simulink model "gm_HFMA_4B_1_5_9_13"  (R2026b)
settings: Solver=FixedStepDiscrete  StopTime=stopTime  FixedStep=1.953125e-06
PreLoadFcn:
  | load('a_luts.mat')
undefined symbols (not defined in the file or in its folder): Ts
libraries: simulink x202, simulink_need_slupdate x99, hdlsllib x91
(part 18 of 20)

== system gm_HFMA_4B_1_5_9_13/Subsystem/HFMA1/crp_temp_shared6/Serializer_Subnetwork1 ==
  in0 : Inport  OutDataTypeStr=fixdt(1,18,0,'DataTypeOverride', 'Off')  PortDimensions=[16]  SampleTime=1.953125e-06
  in1 : Inport  Port=2  OutDataTypeStr=fixdt(0,4,0,'DataTypeOverride', 'Off')  PortDimensions=1  SampleTime=1.953125e-06
  ratechange_splitcomp : Demux  Outputs=16
  splitcomp_multiport : MultiPortSwitch  DataPortOrder=Zero-based contiguous  Inputs=16  DiagnosticForDefault=None  zeroidx=on  OutDataTypeStr=fixdt(1, 18, 0)  SampleTime=1.953125e-06  SaturateOnIntegerOverflow=off  InputSameDT=off
  out0 : Outport  OutDataTypeStr=fixdt(1,18,0,'DataTypeOverride', 'Off')  PortDimensions=1  SampleTime=1.953125e-06
  wires:
  in0/1 -> ratechange_splitcomp/1
  in1/1 -> splitcomp_multiport/1
  ratechange_splitcomp/1 -> splitcomp_multiport/2
  ratechange_splitcomp/2 -> splitcomp_multiport/3
  ratechange_splitcomp/3 -> splitcomp_multiport/4
  ratechange_splitcomp/4 -> splitcomp_multiport/5
  ratechange_splitcomp/7 -> splitcomp_multiport/8
  ratechange_splitcomp/5 -> splitcomp_multiport/6
  ratechange_splitcomp/6 -> splitcomp_multiport/7
  ratechange_splitcomp/8 -> splitcomp_multiport/9
  ratechange_splitcomp/9 -> splitcomp_multiport/10
  ratechange_splitcomp/13 -> splitcomp_multiport/14
  ratechange_splitcomp/12 -> splitcomp_multiport/13
  ratechange_splitcomp/11 -> splitcomp_multiport/12
  ratechange_splitcomp/10 -> splitcomp_multiport/11
  ratechange_splitcomp/16 -> splitcomp_multiport/17
  ratechange_splitcomp/15 -> splitcomp_multiport/16
  ratechange_splitcomp/14 -> splitcomp_multiport/15
  splitcomp_multiport/1 -> out0/1

== system gm_HFMA_4B_1_5_9_13/Subsystem/HFMA1/crp_temp_shared6/counter ==
  globalSchedule : EnablePort  OutDataTypeStr=boolean
  ctr_0_15 : hdlsllib/Sources/HDL Counter  CountType=Count limited  CountInit=0  CountStep=1  CountMax=15  CountFromType=Initial value  CountFrom=0  CountResetPort=off  CountLoadPort=off  CountEnbPort=off  CountDirPort=off  CountHitOutputPort=off  CountDataType=Unsigned  CountWordLen=4  CountFracLen=0  CountSampTime=1.953125e-06
  out0 : Outport  OutDataTypeStr=fixdt(0,4,0,'DataTypeOverride', 'Off')  PortDimensions=1  SampleTime=1.953125e-06  InitialOutput=0
  wires:
  ctr_0_15/1 -> out0/1

== system gm_HFMA_4B_1_5_9_13/Subsystem/HFMA1/crp_temp_shared7/Serializer_Subnetwork ==
  in0 : Inport  OutDataTypeStr=fixdt(1,32,28,'DataTypeOverride', 'Off')  PortDimensions=[2]  SampleTime=1.953125e-06
  in1 : Inport  Port=2  OutDataTypeStr=fixdt(0,1,0,'DataTypeOverride', 'Off')  PortDimensions=1  SampleTime=1.953125e-06
  ratechange_splitcomp : Demux  Outputs=2
  splitcomp_multiport : MultiPortSwitch  DataPortOrder=Zero-based contiguous  Inputs=2  DiagnosticForDefault=None  zeroidx=on  OutDataTypeStr=fixdt(1, 32, 28)  SampleTime=1.953125e-06  SaturateOnIntegerOverflow=off  InputSameDT=off
  out0 : Outport  OutDataTypeStr=fixdt(1,32,28,'DataTypeOverride', 'Off')  PortDimensions=1  SampleTime=1.953125e-06
  wires:
  in0/1 -> ratechange_splitcomp/1
  in1/1 -> splitcomp_multiport/1
  ratechange_splitcomp/2 -> splitcomp_multiport/3
  ratechange_splitcomp/1 -> splitcomp_multiport/2
  splitcomp_multiport/1 -> out0/1

== system gm_HFMA_4B_1_5_9_13/Subsystem/HFMA1/crp_temp_shared7/Serializer_Subnetwork1 ==
  in0 : Inport  OutDataTypeStr=fixdt(1,32,28,'DataTypeOverride', 'Off')  PortDimensions=[2]  SampleTime=1.953125e-06
  in1 : Inport  Port=2  OutDataTypeStr=fixdt(0,1,0,'DataTypeOverride', 'Off')  PortDimensions=1  SampleTime=1.953125e-06
  ratechange_splitcomp : Demux  Outputs=2
  splitcomp_multiport : MultiPortSwitch  DataPortOrder=Zero-based contiguous  Inputs=2  DiagnosticForDefault=None  zeroidx=on  OutDataTypeStr=fixdt(1, 32, 28)  SampleTime=1.953125e-06  SaturateOnIntegerOverflow=off  InputSameDT=off
  out0 : Outport  OutDataTypeStr=fixdt(1,32,28,'DataTypeOverride', 'Off')  PortDimensions=1  SampleTime=1.953125e-06
  wires:
  in1/1 -> splitcomp_multiport/1
  in0/1 -> ratechange_splitcomp/1
  ratechange_splitcomp/2 -> splitcomp_multiport/3
  ratechange_splitcomp/1 -> splitcomp_multiport/2
  splitcomp_multiport/1 -> out0/1

== system gm_HFMA_4B_1_5_9_13/Subsystem/HFMA1/crp_temp_shared7/counter ==
  globalSchedule : EnablePort  OutDataTypeStr=boolean
  ctr_0_1 : hdlsllib/Sources/HDL Counter  CountType=Count limited  CountInit=0  CountStep=1  CountMax=1  CountFromType=Initial value  CountFrom=0  CountResetPort=off  CountLoadPort=off  CountEnbPort=off  CountDirPort=off  CountHitOutputPort=off  CountDataType=Unsigned  CountWordLen=1  CountFracLen=0  CountSampTime=1.953125e-06
  out0 : Outport  OutDataTypeStr=fixdt(0,1,0,'DataTypeOverride', 'Off')  PortDimensions=1  SampleTime=1.953125e-06  InitialOutput=0
  wires:
  ctr_0_1/1 -> out0/1

== system gm_HFMA_4B_1_5_9_13/Subsystem/HFMA1/crp_temp_shared8/Serializer_Subnetwork ==
  in0 : Inport  OutDataTypeStr=fixdt(1,18,0,'DataTypeOverride', 'Off')  PortDimensions=[16]  SampleTime=1.953125e-06
  in1 : Inport  Port=2  OutDataTypeStr=fixdt(0,4,0,'DataTypeOverride', 'Off')  PortDimensions=1  SampleTime=1.953125e-06
  ratechange_splitcomp : Demux  Outputs=16
  splitcomp_multiport : MultiPortSwitch  DataPortOrder=Zero-based contiguous  Inputs=16  DiagnosticForDefault=None  zeroidx=on  OutDataTypeStr=fixdt(1, 18, 0)  SampleTime=1.953125e-06  SaturateOnIntegerOverflow=off  InputSameDT=off
  out0 : Outport  OutDataTypeStr=fixdt(1,18,0,'DataTypeOverride', 'Off')  PortDimensions=1  SampleTime=1.953125e-06
  wires:
  ratechange_splitcomp/16 -> splitcomp_multiport/17
  ratechange_splitcomp/15 -> splitcomp_multiport/16
  ratechange_splitcomp/14 -> splitcomp_multiport/15
  ratechange_splitcomp/13 -> splitcomp_multiport/14
  in0/1 -> ratechange_splitcomp/1
  in1/1 -> splitcomp_multiport/1
  ratechange_splitcomp/1 -> splitcomp_multiport/2
  ratechange_splitcomp/2 -> splitcomp_multiport/3
  ratechange_splitcomp/3 -> splitcomp_multiport/4
  ratechange_splitcomp/4 -> splitcomp_multiport/5
  ratechange_splitcomp/8 -> splitcomp_multiport/9
  ratechange_splitcomp/7 -> splitcomp_multiport/8
  ratechange_splitcomp/5 -> splitcomp_multiport/6
  ratechange_splitcomp/6 -> splitcomp_multiport/7
  ratechange_splitcomp/12 -> splitcomp_multiport/13
  ratechange_splitcomp/11 -> splitcomp_multiport/12
  ratechange_splitcomp/10 -> splitcomp_multiport/11
  ratechange_splitcomp/9 -> splitcomp_multiport/10
  splitcomp_multiport/1 -> out0/1

== system gm_HFMA_4B_1_5_9_13/Subsystem/HFMA1/crp_temp_shared8/Serializer_Subnetwork1 ==
  in0 : Inport  OutDataTypeStr=fixdt(1,18,0,'DataTypeOverride', 'Off')  PortDimensions=[16]  SampleTime=1.953125e-06
  in1 : Inport  Port=2  OutDataTypeStr=fixdt(0,4,0,'DataTypeOverride', 'Off')  PortDimensions=1  SampleTime=1.953125e-06
  ratechange_splitcomp : Demux  Outputs=16
  splitcomp_multiport : MultiPortSwitch  DataPortOrder=Zero-based contiguous  Inputs=16  DiagnosticForDefault=None  zeroidx=on  OutDataTypeStr=fixdt(1, 18, 0)  SampleTime=1.953125e-06  SaturateOnIntegerOverflow=off  InputSameDT=off
  out0 : Outport  OutDataTypeStr=fixdt(1,18,0,'DataTypeOverride', 'Off')  PortDimensions=1  SampleTime=1.953125e-06
  wires:
  in0/1 -> ratechange_splitcomp/1
  in1/1 -> splitcomp_multiport/1
  ratechange_splitcomp/1 -> splitcomp_multiport/2
  ratechange_splitcomp/2 -> splitcomp_multiport/3
  ratechange_splitcomp/3 -> splitcomp_multiport/4
  ratechange_splitcomp/4 -> splitcomp_multiport/5
  ratechange_splitcomp/5 -> splitcomp_multiport/6
  ratechange_splitcomp/7 -> splitcomp_multiport/8
  ratechange_splitcomp/6 -> splitcomp_multiport/7
  ratechange_splitcomp/8 -> splitcomp_multiport/9
  ratechange_splitcomp/16 -> splitcomp_multiport/17
  ratechange_splitcomp/15 -> splitcomp_multiport/16
  ratechange_splitcomp/9 -> splitcomp_multiport/10
  ratechange_splitcomp/10 -> splitcomp_multiport/11
  ratechange_splitcomp/14 -> splitcomp_multiport/15
  ratechange_splitcomp/13 -> splitcomp_multiport/14
  ratechange_splitcomp/12 -> splitcomp_multiport/13
  ratechange_splitcomp/11 -> splitcomp_multiport/12
  splitcomp_multiport/1 -> out0/1

== system gm_HFMA_4B_1_5_9_13/Subsystem/HFMA1/crp_temp_shared8/counter ==
  globalSchedule : EnablePort  OutDataTypeStr=boolean
  ctr_0_15 : hdlsllib/Sources/HDL Counter  CountType=Count limited  CountInit=0  CountStep=1  CountMax=15  CountFromType=Initial value  CountFrom=0  CountResetPort=off  CountLoadPort=off  CountEnbPort=off  CountDirPort=off  CountHitOutputPort=off  CountDataType=Unsigned  CountWordLen=4  CountFracLen=0  CountSampTime=1.953125e-06
  out0 : Outport  OutDataTypeStr=fixdt(0,4,0,'DataTypeOverride', 'Off')  PortDimensions=1  SampleTime=1.953125e-06  InitialOutput=0
  wires:
  ctr_0_15/1 -> out0/1

== system gm_HFMA_4B_1_5_9_13/Subsystem/HFMA1/crp_temp_shared9/Serializer_Subnetwork ==
  in0 : Inport  OutDataTypeStr=fixdt(1,18,16,'DataTypeOverride', 'Off')  PortDimensions=[2]  SampleTime=1.953125e-06
  in1 : Inport  Port=2  OutDataTypeStr=fixdt(0,1,0,'DataTypeOverride', 'Off')  PortDimensions=1  SampleTime=1.953125e-06
  ratechange_splitcomp : Demux  Outputs=2
  splitcomp_multiport : MultiPortSwitch  DataPortOrder=Zero-based contiguous  Inputs=2  DiagnosticForDefault=None  zeroidx=on  OutDataTypeStr=fixdt(1, 18, 16)  SampleTime=1.953125e-06  SaturateOnIntegerOverflow=off  InputSameDT=off
  out0 : Outport  OutDataTypeStr=fixdt(1,18,16,'DataTypeOverride', 'Off')  PortDimensions=1  SampleTime=1.953125e-06
  wires:
  in0/1 -> ratechange_splitcomp/1
  in1/1 -> splitcomp_multiport/1
  ratechange_splitcomp/2 -> splitcomp_multiport/3
  ratechange_splitcomp/1 -> splitcomp_multiport/2
  splitcomp_multiport/1 -> out0/1

== system gm_HFMA_4B_1_5_9_13/Subsystem/HFMA1/crp_temp_shared9/Serializer_Subnetwork1 ==
  in0 : Inport  OutDataTypeStr=fixdt(1,18,16,'DataTypeOverride', 'Off')  PortDimensions=[2]  SampleTime=1.953125e-06
  in1 : Inport  Port=2  OutDataTypeStr=fixdt(0,1,0,'DataTypeOverride', 'Off')  PortDimensions=1  SampleTime=1.953125e-06
  ratechange_splitcomp : Demux  Outputs=2
  splitcomp_multiport : MultiPortSwitch  DataPortOrder=Zero-based contiguous  Inputs=2  DiagnosticForDefault=None  zeroidx=on  OutDataTypeStr=fixdt(1, 18, 16)  SampleTime=1.953125e-06  SaturateOnIntegerOverflow=off  InputSameDT=off
  out0 : Outport  OutDataTypeStr=fixdt(1,18,16,'DataTypeOverride', 'Off')  PortDimensions=1  SampleTime=1.953125e-06
  wires:
  in0/1 -> ratechange_splitcomp/1
  in1/1 -> splitcomp_multiport/1
  ratechange_splitcomp/2 -> splitcomp_multiport/3
  ratechange_splitcomp/1 -> splitcomp_multiport/2
  splitcomp_multiport/1 -> out0/1

== system gm_HFMA_4B_1_5_9_13/Subsystem/HFMA1/crp_temp_shared9/counter ==
  globalSchedule : EnablePort  OutDataTypeStr=boolean
  ctr_0_1 : hdlsllib/Sources/HDL Counter  CountType=Count limited  CountInit=0  CountStep=1  CountMax=1  CountFromType=Initial value  CountFrom=0  CountResetPort=off  CountLoadPort=off  CountEnbPort=off  CountDirPort=off  CountHitOutputPort=off  CountDataType=Unsigned  CountWordLen=1  CountFracLen=0  CountSampTime=1.953125e-06
  out0 : Outport  OutDataTypeStr=fixdt(0,1,0,'DataTypeOverride', 'Off')  PortDimensions=1  SampleTime=1.953125e-06  InitialOutput=0
  wires:
  ctr_0_1/1 -> out0/1

== system gm_HFMA_4B_1_5_9_13/Subsystem/HFMA13/crp_temp_shared/Product3_out1_bypass ==
  in0 : Inport  OutDataTypeStr=fixdt(1,51,0,'DataTypeOverride', 'Off')  PortDimensions=1  SampleTime=1.953125e-06
  in1 : Inport  Port=2  OutDataTypeStr=boolean  PortDimensions=1  SampleTime=1.953125e-06
  Product3_out1_enb : Switch  Criteria=u2 ~= 0  OutDataTypeStr=fixdt(1, 51, 0)  SampleTime=1.953125e-06  SaturateOnIntegerOverflow=off  InputSameDT=off
  Product3_out1_state : Delay  DelayLength=1  InitialCondition=0  SampleTime=1.953125e-06
  out0 : Outport  OutDataTypeStr=fixdt(1,51,0,'DataTypeOverride', 'Off')  PortDimensions=1  SampleTime=1.953125e-06
  wires:
  in0/1 -> Product3_out1_enb/1
  in1/1 -> Product3_out1_enb/2
  Product3_out1_enb/1 -> Product3_out1_state/1, out0/1
  Product3_out1_state/1 -> Product3_out1_enb/3

== system gm_HFMA_4B_1_5_9_13/Subsystem/HFMA13/crp_temp_shared/Serializer_Subnetwork ==
  in0 : Inport  OutDataTypeStr=fixdt(1,19,0,'DataTypeOverride', 'Off')  PortDimensions=[15]  SampleTime=1.953125e-06
  in1 : Inport  Port=2  OutDataTypeStr=fixdt(0,4,0,'DataTypeOverride', 'Off')  PortDimensions=1  SampleTime=1.953125e-06
  ratechange_splitcomp : Demux  Outputs=15
  splitcomp_multiport : MultiPortSwitch  DataPortOrder=Zero-based contiguous  Inputs=15  DiagnosticForDefault=None  zeroidx=on  OutDataTypeStr=fixdt(1, 19, 0)  SampleTime=1.953125e-06  SaturateOnIntegerOverflow=off  InputSameDT=off
  out0 : Outport  OutDataTypeStr=fixdt(1,19,0,'DataTypeOverride', 'Off')  PortDimensions=1  SampleTime=1.953125e-06
  wires:
  in0/1 -> ratechange_splitcomp/1
  in1/1 -> splitcomp_multiport/1
  ratechange_splitcomp/8 -> splitcomp_multiport/9
  ratechange_splitcomp/2 -> splitcomp_multiport/3
  ratechange_splitcomp/4 -> splitcomp_multiport/5
  ratechange_splitcomp/6 -> splitcomp_multiport/7
  ratechange_splitcomp/7 -> splitcomp_multiport/8
  ratechange_splitcomp/1 -> splitcomp_multiport/2
  ratechange_splitcomp/3 -> splitcomp_multiport/4
  ratechange_splitcomp/5 -> splitcomp_multiport/6
  ratechange_splitcomp/15 -> splitcomp_multiport/16
  ratechange_splitcomp/13 -> splitcomp_multiport/14
  ratechange_splitcomp/11 -> splitcomp_multiport/12
  ratechange_splitcomp/9 -> splitcomp_multiport/10
  ratechange_splitcomp/14 -> splitcomp_multiport/15
  ratechange_splitcomp/12 -> splitcomp_multiport/13
  ratechange_splitcomp/10 -> splitcomp_multiport/11
  splitcomp_multiport/1 -> out0/1

== system gm_HFMA_4B_1_5_9_13/Subsystem/HFMA13/crp_temp_shared/Serializer_Subnetwork1 ==
  in0 : Inport  OutDataTypeStr=fixdt(1,33,0,'DataTypeOverride', 'Off')  PortDimensions=[15]  SampleTime=1.953125e-06
  in1 : Inport  Port=2  OutDataTypeStr=fixdt(0,4,0,'DataTypeOverride', 'Off')  PortDimensions=1  SampleTime=1.953125e-06
  ratechange_splitcomp : Demux  Outputs=15
  splitcomp_multiport : MultiPortSwitch  DataPortOrder=Zero-based contiguous  Inputs=15  DiagnosticForDefault=None  zeroidx=on  OutDataTypeStr=fixdt(1, 33, 0)  SampleTime=1.953125e-06  SaturateOnIntegerOverflow=off  InputSameDT=off
  out0 : Outport  OutDataTypeStr=fixdt(1,33,0,'DataTypeOverride', 'Off')  PortDimensions=1  SampleTime=1.953125e-06
  wires:
  in1/1 -> splitcomp_multiport/1
  in0/1 -> ratechange_splitcomp/1
  ratechange_splitcomp/1 -> splitcomp_multiport/2
  ratechange_splitcomp/3 -> splitcomp_multiport/4
  ratechange_splitcomp/2 -> splitcomp_multiport/3
  ratechange_splitcomp/4 -> splitcomp_multiport/5
  ratechange_splitcomp/6 -> splitcomp_multiport/7
  ratechange_splitcomp/5 -> splitcomp_multiport/6
  ratechange_splitcomp/7 -> splitcomp_multiport/8
  ratechange_splitcomp/8 -> splitcomp_multiport/9
  ratechange_splitcomp/9 -> splitcomp_multiport/10
  ratechange_splitcomp/14 -> splitcomp_multiport/15
  ratechange_splitcomp/12 -> splitcomp_multiport/13
  ratechange_splitcomp/10 -> splitcomp_multiport/11
  ratechange_splitcomp/15 -> splitcomp_multiport/16
  ratechange_splitcomp/13 -> splitcomp_multiport/14
  ratechange_splitcomp/11 -> splitcomp_multiport/12
  splitcomp_multiport/1 -> out0/1

== system gm_HFMA_4B_1_5_9_13/Subsystem/HFMA13/crp_temp_shared/counter ==
  globalSchedule : EnablePort  OutDataTypeStr=boolean
  ctr_0_14 : hdlsllib/Sources/HDL Counter  CountType=Count limited  CountInit=0  CountStep=1  CountMax=14  CountFromType=Initial value  CountFrom=0  CountResetPort=off  CountLoadPort=off  CountEnbPort=off  CountDirPort=off  CountHitOutputPort=off  CountDataType=Unsigned  CountWordLen=4  CountFracLen=0  CountSampTime=1.953125e-06
  out0 : Outport  OutDataTypeStr=fixdt(0,4,0,'DataTypeOverride', 'Off')  PortDimensions=1  SampleTime=1.953125e-06  InitialOutput=0
  wires:
  ctr_0_14/1 -> out0/1

== system gm_HFMA_4B_1_5_9_13/Subsystem/HFMA13/crp_temp_shared/sharing_subsystem ==
  in0 : Inport  OutDataTypeStr=fixdt(1,33,0,'DataTypeOverride', 'Off')  PortDimensions=1  SampleTime=1.953125e-06
  in1 : Inport  Port=2  OutDataTypeStr=fixdt(1,19,0,'DataTypeOverride', 'Off')  PortDimensions=1  SampleTime=1.953125e-06
  Product : Product  Inputs=**  OutDataTypeStr=fixdt(1, 51, 0)  SampleTime=1.953125e-06
  out0 : Outport  OutDataTypeStr=fixdt(1,51,0,'DataTypeOverride', 'Off')  PortDimensions=1  SampleTime=1.953125e-06
  wires:
  in1/1 -> Product/2
  in0/1 -> Product/1
  Product/1 -> out0/1

== system gm_HFMA_4B_1_5_9_13/Subsystem/HFMA13/crp_temp_shared1/Serializer_Subnetwork ==
  in0 : Inport  OutDataTypeStr=fixdt(1,20,17,'DataTypeOverride', 'Off')  PortDimensions=[8]  SampleTime=1.953125e-06
  in1 : Inport  Port=2  OutDataTypeStr=fixdt(0,3,0,'DataTypeOverride', 'Off')  PortDimensions=1  SampleTime=1.953125e-06
  ratechange_splitcomp : Demux  Outputs=8
  splitcomp_multiport : MultiPortSwitch  DataPortOrder=Zero-based contiguous  Inputs=8  DiagnosticForDefault=None  zeroidx=on  OutDataTypeStr=fixdt(1, 20, 17)  SampleTime=1.953125e-06  SaturateOnIntegerOverflow=off  InputSameDT=off
  out0 : Outport  OutDataTypeStr=fixdt(1,20,17,'DataTypeOverride', 'Off')  PortDimensions=1  SampleTime=1.953125e-06
  wires:
  in0/1 -> ratechange_splitcomp/1
  ratechange_splitcomp/1 -> splitcomp_multiport/2
  in1/1 -> splitcomp_multiport/1
  ratechange_splitcomp/8 -> splitcomp_multiport/9
  ratechange_splitcomp/2 -> splitcomp_multiport/3
  ratechange_splitcomp/4 -> splitcomp_multiport/5
  ratechange_splitcomp/6 -> splitcomp_multiport/7
  ratechange_splitcomp/7 -> splitcomp_multiport/8
  ratechange_splitcomp/3 -> splitcomp_multiport/4
  ratechange_splitcomp/5 -> splitcomp_multiport/6
  splitcomp_multiport/1 -> out0/1

== system gm_HFMA_4B_1_5_9_13/Subsystem/HFMA13/crp_temp_shared1/Serializer_Subnetwork1 ==
  in0 : Inport  OutDataTypeStr=fixdt(1,18,16,'DataTypeOverride', 'Off')  PortDimensions=[8]  SampleTime=1.953125e-06
  in1 : Inport  Port=2  OutDataTypeStr=fixdt(0,3,0,'DataTypeOverride', 'Off')  PortDimensions=1  SampleTime=1.953125e-06
  ratechange_splitcomp : Demux  Outputs=8
  splitcomp_multiport : MultiPortSwitch  DataPortOrder=Zero-based contiguous  Inputs=8  DiagnosticForDefault=None  zeroidx=on  OutDataTypeStr=fixdt(1, 18, 16)  SampleTime=1.953125e-06  SaturateOnIntegerOverflow=off  InputSameDT=off
  out0 : Outport  OutDataTypeStr=fixdt(1,18,16,'DataTypeOverride', 'Off')  PortDimensions=1  SampleTime=1.953125e-06
  wires:
  ratechange_splitcomp/2 -> splitcomp_multiport/3
  ratechange_splitcomp/4 -> splitcomp_multiport/5
  ratechange_splitcomp/6 -> splitcomp_multiport/7
  ratechange_splitcomp/7 -> splitcomp_multiport/8
  ratechange_splitcomp/3 -> splitcomp_multiport/4
  ratechange_splitcomp/5 -> splitcomp_multiport/6
  in1/1 -> splitcomp_multiport/1
  in0/1 -> ratechange_splitcomp/1
  ratechange_splitcomp/1 -> splitcomp_multiport/2
  splitcomp_multiport/1 -> out0/1
  ratechange_splitcomp/8 -> splitcomp_multiport/9

== system gm_HFMA_4B_1_5_9_13/Subsystem/HFMA13/crp_temp_shared1/counter ==
  globalSchedule : EnablePort  OutDataTypeStr=boolean
  ctr_0_7 : hdlsllib/Sources/HDL Counter  CountType=Count limited  CountInit=0  CountStep=1  CountMax=7  CountFromType=Initial value  CountFrom=0  CountResetPort=off  CountLoadPort=off  CountEnbPort=off  CountDirPort=off  CountHitOutputPort=off  CountDataType=Unsigned  CountWordLen=3  CountFracLen=0  CountSampTime=1.953125e-06
  out0 : Outport  OutDataTypeStr=fixdt(0,3,0,'DataTypeOverride', 'Off')  PortDimensions=1  SampleTime=1.953125e-06  InitialOutput=0
  wires:
  ctr_0_7/1 -> out0/1

== system gm_HFMA_4B_1_5_9_13/Subsystem/HFMA13/crp_temp_shared2/Serializer_Subnetwork ==
  in0 : Inport  OutDataTypeStr=fixdt(1,18,0,'DataTypeOverride', 'Off')  PortDimensions=[16]  SampleTime=1.953125e-06
  in1 : Inport  Port=2  OutDataTypeStr=fixdt(0,4,0,'DataTypeOverride', 'Off')  PortDimensions=1  SampleTime=1.953125e-06
  ratechange_splitcomp : Demux  Outputs=16
  splitcomp_multiport : MultiPortSwitch  DataPortOrder=Zero-based contiguous  Inputs=16  DiagnosticForDefault=None  zeroidx=on  OutDataTypeStr=fixdt(1, 18, 0)  SampleTime=1.953125e-06  SaturateOnIntegerOverflow=off  InputSameDT=off
  out0 : Outport  OutDataTypeStr=fixdt(1,18,0,'DataTypeOverride', 'Off')  PortDimensions=1  SampleTime=1.953125e-06
  wires:
  in0/1 -> ratechange_splitcomp/1
  ratechange_splitcomp/1 -> splitcomp_multiport/2
  in1/1 -> splitcomp_multiport/1
  ratechange_splitcomp/8 -> splitcomp_multiport/9
  ratechange_splitcomp/2 -> splitcomp_multiport/3
  ratechange_splitcomp/4 -> splitcomp_multiport/5
  ratechange_splitcomp/6 -> splitcomp_multiport/7
  ratechange_splitcomp/9 -> splitcomp_multiport/10
  ratechange_splitcomp/7 -> splitcomp_multiport/8
  ratechange_splitcomp/3 -> splitcomp_multiport/4
  ratechange_splitcomp/5 -> splitcomp_multiport/6
  ratechange_splitcomp/16 -> splitcomp_multiport/17
  ratechange_splitcomp/14 -> splitcomp_multiport/15
  ratechange_splitcomp/12 -> splitcomp_multiport/13
  ratechange_splitcomp/10 -> splitcomp_multiport/11
  ratechange_splitcomp/15 -> splitcomp_multiport/16
  ratechange_splitcomp/13 -> splitcomp_multiport/14
  ratechange_splitcomp/11 -> splitcomp_multiport/12
  splitcomp_multiport/1 -> out0/1

== system gm_HFMA_4B_1_5_9_13/Subsystem/HFMA13/crp_temp_shared2/Serializer_Subnetwork1 ==
  in0 : Inport  OutDataTypeStr=fixdt(1,18,0,'DataTypeOverride', 'Off')  PortDimensions=[16]  SampleTime=1.953125e-06
  in1 : Inport  Port=2  OutDataTypeStr=fixdt(0,4,0,'DataTypeOverride', 'Off')  PortDimensions=1  SampleTime=1.953125e-06
  ratechange_splitcomp : Demux  Outputs=16
  splitcomp_multiport : MultiPortSwitch  DataPortOrder=Zero-based contiguous  Inputs=16  DiagnosticForDefault=None  zeroidx=on  OutDataTypeStr=fixdt(1, 18, 0)  SampleTime=1.953125e-06  SaturateOnIntegerOverflow=off  InputSameDT=off
  out0 : Outport  OutDataTypeStr=fixdt(1,18,0,'DataTypeOverride', 'Off')  PortDimensions=1  SampleTime=1.953125e-06
  wires:
  in0/1 -> ratechange_splitcomp/1
  in1/1 -> splitcomp_multiport/1
  ratechange_splitcomp/5 -> splitcomp_multiport/6
  ratechange_splitcomp/2 -> splitcomp_multiport/3
  ratechange_splitcomp/4 -> splitcomp_multiport/5
  ratechange_splitcomp/1 -> splitcomp_multiport/2
  ratechange_splitcomp/3 -> splitcomp_multiport/4
  ratechange_splitcomp/6 -> splitcomp_multiport/7
  ratechange_splitcomp/11 -> splitcomp_multiport/12
  ratechange_splitcomp/9 -> splitcomp_multiport/10
  ratechange_splitcomp/7 -> splitcomp_multiport/8
  ratechange_splitcomp/12 -> splitcomp_multiport/13
  ratechange_splitcomp/10 -> splitcomp_multiport/11
  ratechange_splitcomp/8 -> splitcomp_multiport/9
  ratechange_splitcomp/15 -> splitcomp_multiport/16
  ratechange_splitcomp/13 -> splitcomp_multiport/14
  ratechange_splitcomp/16 -> splitcomp_multiport/17
  ratechange_splitcomp/14 -> splitcomp_multiport/15
  splitcomp_multiport/1 -> out0/1

== system gm_HFMA_4B_1_5_9_13/Subsystem/HFMA13/crp_temp_shared2/counter ==
  globalSchedule : EnablePort  OutDataTypeStr=boolean
  ctr_0_15 : hdlsllib/Sources/HDL Counter  CountType=Count limited  CountInit=0  CountStep=1  CountMax=15  CountFromType=Initial value  CountFrom=0  CountResetPort=off  CountLoadPort=off  CountEnbPort=off  CountDirPort=off  CountHitOutputPort=off  CountDataType=Unsigned  CountWordLen=4  CountFracLen=0  CountSampTime=1.953125e-06
  out0 : Outport  OutDataTypeStr=fixdt(0,4,0,'DataTypeOverride', 'Off')  PortDimensions=1  SampleTime=1.953125e-06  InitialOutput=0
  wires:
  ctr_0_15/1 -> out0/1

== system gm_HFMA_4B_1_5_9_13/Subsystem/HFMA13/crp_temp_shared3/Serializer_Subnetwork ==
  in0 : Inport  OutDataTypeStr=fixdt(1,18,0,'DataTypeOverride', 'Off')  PortDimensions=[16]  SampleTime=1.953125e-06
  in1 : Inport  Port=2  OutDataTypeStr=fixdt(0,4,0,'DataTypeOverride', 'Off')  PortDimensions=1  SampleTime=1.953125e-06
  ratechange_splitcomp : Demux  Outputs=16
  splitcomp_multiport : MultiPortSwitch  DataPortOrder=Zero-based contiguous  Inputs=16  DiagnosticForDefault=None  zeroidx=on  OutDataTypeStr=fixdt(1, 18, 0)  SampleTime=1.953125e-06  SaturateOnIntegerOverflow=off  InputSameDT=off
  out0 : Outport  OutDataTypeStr=fixdt(1,18,0,'DataTypeOverride', 'Off')  PortDimensions=1  SampleTime=1.953125e-06
  wires:
  in0/1 -> ratechange_splitcomp/1
  in1/1 -> splitcomp_multiport/1
  ratechange_splitcomp/1 -> splitcomp_multiport/2
  ratechange_splitcomp/3 -> splitcomp_multiport/4
  ratechange_splitcomp/2 -> splitcomp_multiport/3
  ratechange_splitcomp/10 -> splitcomp_multiport/11
  ratechange_splitcomp/8 -> splitcomp_multiport/9
  ratechange_splitcomp/4 -> splitcomp_multiport/5
  ratechange_splitcomp/6 -> splitcomp_multiport/7
  ratechange_splitcomp/11 -> splitcomp_multiport/12
  ratechange_splitcomp/9 -> splitcomp_multiport/10
  ratechange_splitcomp/7 -> splitcomp_multiport/8
  ratechange_splitcomp/5 -> splitcomp_multiport/6
  ratechange_splitcomp/16 -> splitcomp_multiport/17
  ratechange_splitcomp/14 -> splitcomp_multiport/15
  ratechange_splitcomp/12 -> splitcomp_multiport/13
  ratechange_splitcomp/15 -> splitcomp_multiport/16
  ratechange_splitcomp/13 -> splitcomp_multiport/14
  splitcomp_multiport/1 -> out0/1

== system gm_HFMA_4B_1_5_9_13/Subsystem/HFMA13/crp_temp_shared3/Serializer_Subnetwork1 ==
  in0 : Inport  OutDataTypeStr=fixdt(1,18,0,'DataTypeOverride', 'Off')  PortDimensions=[16]  SampleTime=1.953125e-06
  in1 : Inport  Port=2  OutDataTypeStr=fixdt(0,4,0,'DataTypeOverride', 'Off')  PortDimensions=1  SampleTime=1.953125e-06
  ratechange_splitcomp : Demux  Outputs=16
  splitcomp_multiport : MultiPortSwitch  DataPortOrder=Zero-based contiguous  Inputs=16  DiagnosticForDefault=None  zeroidx=on  OutDataTypeStr=fixdt(1, 18, 0)  SampleTime=1.953125e-06  SaturateOnIntegerOverflow=off  InputSameDT=off
  out0 : Outport  OutDataTypeStr=fixdt(1,18,0,'DataTypeOverride', 'Off')  PortDimensions=1  SampleTime=1.953125e-06
  wires:
  in0/1 -> ratechange_splitcomp/1
  splitcomp_multiport/1 -> out0/1
  ratechange_splitcomp/16 -> splitcomp_multiport/17
  ratechange_splitcomp/1 -> splitcomp_multiport/2
  ratechange_splitcomp/15 -> splitcomp_multiport/16
  in1/1 -> splitcomp_multiport/1
  ratechange_splitcomp/6 -> splitcomp_multiport/7
  ratechange_splitcomp/2 -> splitcomp_multiport/3
  ratechange_splitcomp/4 -> splitcomp_multiport/5
  ratechange_splitcomp/3 -> splitcomp_multiport/4
  ratechange_splitcomp/5 -> splitcomp_multiport/6
  ratechange_splitcomp/13 -> splitcomp_multiport/14
  ratechange_splitcomp/11 -> splitcomp_multiport/12
  ratechange_splitcomp/9 -> splitcomp_multiport/10
  ratechange_splitcomp/7 -> splitcomp_multiport/8
  ratechange_splitcomp/14 -> splitcomp_multiport/15
  ratechange_splitcomp/12 -> splitcomp_multiport/13
  ratechange_splitcomp/10 -> splitcomp_multiport/11
  ratechange_splitcomp/8 -> splitcomp_multiport/9

== system gm_HFMA_4B_1_5_9_13/Subsystem/HFMA13/crp_temp_shared3/counter ==
  globalSchedule : EnablePort  OutDataTypeStr=boolean
  ctr_0_15 : hdlsllib/Sources/HDL Counter  CountType=Count limited  CountInit=0  CountStep=1  CountMax=15  CountFromType=Initial value  CountFrom=0  CountResetPort=off  CountLoadPort=off  CountEnbPort=off  CountDirPort=off  CountHitOutputPort=off  CountDataType=Unsigned  CountWordLen=4  CountFracLen=0  CountSampTime=1.953125e-06
  out0 : Outport  OutDataTypeStr=fixdt(0,4,0,'DataTypeOverride', 'Off')  PortDimensions=1  SampleTime=1.953125e-06  InitialOutput=0
  wires:
  ctr_0_15/1 -> out0/1

== system gm_HFMA_4B_1_5_9_13/Subsystem/HFMA13/crp_temp_shared4/Serializer_Subnetwork ==
  in0 : Inport  OutDataTypeStr=fixdt(1,18,0,'DataTypeOverride', 'Off')  PortDimensions=[16]  SampleTime=1.953125e-06
  in1 : Inport  Port=2  OutDataTypeStr=fixdt(0,4,0,'DataTypeOverride', 'Off')  PortDimensions=1  SampleTime=1.953125e-06
  ratechange_splitcomp : Demux  Outputs=16
  splitcomp_multiport : MultiPortSwitch  DataPortOrder=Zero-based contiguous  Inputs=16  DiagnosticForDefault=None  zeroidx=on  OutDataTypeStr=fixdt(1, 18, 0)  SampleTime=1.953125e-06  SaturateOnIntegerOverflow=off  InputSameDT=off
  out0 : Outport  OutDataTypeStr=fixdt(1,18,0,'DataTypeOverride', 'Off')  PortDimensions=1  SampleTime=1.953125e-06
  wires:
  in0/1 -> ratechange_splitcomp/1
  ratechange_splitcomp/1 -> splitcomp_multiport/2
  in1/1 -> splitcomp_multiport/1
  ratechange_splitcomp/8 -> splitcomp_multiport/9
  ratechange_splitcomp/2 -> splitcomp_multiport/3
  ratechange_splitcomp/4 -> splitcomp_multiport/5
  ratechange_splitcomp/6 -> splitcomp_multiport/7
  ratechange_splitcomp/9 -> splitcomp_multiport/10
  ratechange_splitcomp/7 -> splitcomp_multiport/8
  ratechange_splitcomp/3 -> splitcomp_multiport/4
  ratechange_splitcomp/5 -> splitcomp_multiport/6
  ratechange_splitcomp/16 -> splitcomp_multiport/17
  ratechange_splitcomp/14 -> splitcomp_multiport/15
  ratechange_splitcomp/12 -> splitcomp_multiport/13
  ratechange_splitcomp/10 -> splitcomp_multiport/11
  ratechange_splitcomp/15 -> splitcomp_multiport/16
  ratechange_splitcomp/13 -> splitcomp_multiport/14
  ratechange_splitcomp/11 -> splitcomp_multiport/12
  splitcomp_multiport/1 -> out0/1

== system gm_HFMA_4B_1_5_9_13/Subsystem/HFMA13/crp_temp_shared4/Serializer_Subnetwork1 ==
  in0 : Inport  OutDataTypeStr=fixdt(1,18,0,'DataTypeOverride', 'Off')  PortDimensions=[16]  SampleTime=1.953125e-06
  in1 : Inport  Port=2  OutDataTypeStr=fixdt(0,4,0,'DataTypeOverride', 'Off')  PortDimensions=1  SampleTime=1.953125e-06
  ratechange_splitcomp : Demux  Outputs=16
  splitcomp_multiport : MultiPortSwitch  DataPortOrder=Zero-based contiguous  Inputs=16  DiagnosticForDefault=None  zeroidx=on  OutDataTypeStr=fixdt(1, 18, 0)  SampleTime=1.953125e-06  SaturateOnIntegerOverflow=off  InputSameDT=off
  out0 : Outport  OutDataTypeStr=fixdt(1,18,0,'DataTypeOverride', 'Off')  PortDimensions=1  SampleTime=1.953125e-06
  wires:
  ratechange_splitcomp/5 -> splitcomp_multiport/6
  in0/1 -> ratechange_splitcomp/1
  in1/1 -> splitcomp_multiport/1
  ratechange_splitcomp/2 -> splitcomp_multiport/3
  ratechange_splitcomp/4 -> splitcomp_multiport/5
  ratechange_splitcomp/1 -> splitcomp_multiport/2
  ratechange_splitcomp/3 -> splitcomp_multiport/4
  ratechange_splitcomp/6 -> splitcomp_multiport/7
  ratechange_splitcomp/11 -> splitcomp_multiport/12
  ratechange_splitcomp/9 -> splitcomp_multiport/10
  ratechange_splitcomp/7 -> splitcomp_multiport/8
  ratechange_splitcomp/12 -> splitcomp_multiport/13
  ratechange_splitcomp/10 -> splitcomp_multiport/11
  ratechange_splitcomp/8 -> splitcomp_multiport/9
  ratechange_splitcomp/15 -> splitcomp_multiport/16
  ratechange_splitcomp/13 -> splitcomp_multiport/14
  ratechange_splitcomp/16 -> splitcomp_multiport/17
  ratechange_splitcomp/14 -> splitcomp_multiport/15
  splitcomp_multiport/1 -> out0/1

== system gm_HFMA_4B_1_5_9_13/Subsystem/HFMA13/crp_temp_shared4/counter ==
  globalSchedule : EnablePort  OutDataTypeStr=boolean
  ctr_0_15 : hdlsllib/Sources/HDL Counter  CountType=Count limited  CountInit=0  CountStep=1  CountMax=15  CountFromType=Initial value  CountFrom=0  CountResetPort=off  CountLoadPort=off  CountEnbPort=off  CountDirPort=off  CountHitOutputPort=off  CountDataType=Unsigned  CountWordLen=4  CountFracLen=0  CountSampTime=1.953125e-06
  out0 : Outport  OutDataTypeStr=fixdt(0,4,0,'DataTypeOverride', 'Off')  PortDimensions=1  SampleTime=1.953125e-06  InitialOutput=0
  wires:
  ctr_0_15/1 -> out0/1

== system gm_HFMA_4B_1_5_9_13/Subsystem/HFMA13/crp_temp_shared5/Serializer_Subnetwork ==
  in0 : Inport  OutDataTypeStr=fixdt(1,18,0,'DataTypeOverride', 'Off')  PortDimensions=[16]  SampleTime=1.953125e-06
  in1 : Inport  Port=2  OutDataTypeStr=fixdt(0,4,0,'DataTypeOverride', 'Off')  PortDimensions=1  SampleTime=1.953125e-06
  ratechange_splitcomp : Demux  Outputs=16
  splitcomp_multiport : MultiPortSwitch  DataPortOrder=Zero-based contiguous  Inputs=16  DiagnosticForDefault=None  zeroidx=on  OutDataTypeStr=fixdt(1, 18, 0)  SampleTime=1.953125e-06  SaturateOnIntegerOverflow=off  InputSameDT=off
  out0 : Outport  OutDataTypeStr=fixdt(1,18,0,'DataTypeOverride', 'Off')  PortDimensions=1  SampleTime=1.953125e-06
  wires:
  in0/1 -> ratechange_splitcomp/1
  in1/1 -> splitcomp_multiport/1
  ratechange_splitcomp/2 -> splitcomp_multiport/3
  ratechange_splitcomp/4 -> splitcomp_multiport/5
  ratechange_splitcomp/1 -> splitcomp_multiport/2
  ratechange_splitcomp/3 -> splitcomp_multiport/4
  ratechange_splitcomp/12 -> splitcomp_multiport/13
  ratechange_splitcomp/10 -> splitcomp_multiport/11
  ratechange_splitcomp/8 -> splitcomp_multiport/9
  ratechange_splitcomp/6 -> splitcomp_multiport/7
  ratechange_splitcomp/11 -> splitcomp_multiport/12
  ratechange_splitcomp/9 -> splitcomp_multiport/10
  ratechange_splitcomp/7 -> splitcomp_multiport/8
  ratechange_splitcomp/5 -> splitcomp_multiport/6
  ratechange_splitcomp/15 -> splitcomp_multiport/16
  ratechange_splitcomp/13 -> splitcomp_multiport/14
  ratechange_splitcomp/16 -> splitcomp_multiport/17
  ratechange_splitcomp/14 -> splitcomp_multiport/15
  splitcomp_multiport/1 -> out0/1

== system gm_HFMA_4B_1_5_9_13/Subsystem/HFMA13/crp_temp_shared5/Serializer_Subnetwork1 ==
  in0 : Inport  OutDataTypeStr=fixdt(1,18,0,'DataTypeOverride', 'Off')  PortDimensions=[16]  SampleTime=1.953125e-06
  in1 : Inport  Port=2  OutDataTypeStr=fixdt(0,4,0,'DataTypeOverride', 'Off')  PortDimensions=1  SampleTime=1.953125e-06
  ratechange_splitcomp : Demux  Outputs=16
  splitcomp_multiport : MultiPortSwitch  DataPortOrder=Zero-based contiguous  Inputs=16  DiagnosticForDefault=None  zeroidx=on  OutDataTypeStr=fixdt(1, 18, 0)  SampleTime=1.953125e-06  SaturateOnIntegerOverflow=off  InputSameDT=off
  out0 : Outport  OutDataTypeStr=fixdt(1,18,0,'DataTypeOverride', 'Off')  PortDimensions=1  SampleTime=1.953125e-06
  wires:
  in1/1 -> splitcomp_multiport/1
  in0/1 -> ratechange_splitcomp/1
  ratechange_splitcomp/2 -> splitcomp_multiport/3
  ratechange_splitcomp/1 -> splitcomp_multiport/2
  ratechange_splitcomp/4 -> splitcomp_multiport/5
  ratechange_splitcomp/6 -> splitcomp_multiport/7
  ratechange_splitcomp/3 -> splitcomp_multiport/4
  ratechange_splitcomp/5 -> splitcomp_multiport/6
  ratechange_splitcomp/7 -> splitcomp_multiport/8
  ratechange_splitcomp/14 -> splitcomp_multiport/15
  ratechange_splitcomp/12 -> splitcomp_multiport/13
  ratechange_splitcomp/10 -> splitcomp_multiport/11
  ratechange_splitcomp/8 -> splitcomp_multiport/9
  ratechange_splitcomp/15 -> splitcomp_multiport/16
  ratechange_splitcomp/13 -> splitcomp_multiport/14
  ratechange_splitcomp/11 -> splitcomp_multiport/12
  ratechange_splitcomp/9 -> splitcomp_multiport/10
  splitcomp_multiport/1 -> out0/1
  ratechange_splitcomp/16 -> splitcomp_multiport/17

== system gm_HFMA_4B_1_5_9_13/Subsystem/HFMA13/crp_temp_shared5/counter ==
  globalSchedule : EnablePort  OutDataTypeStr=boolean
  ctr_0_15 : hdlsllib/Sources/HDL Counter  CountType=Count limited  CountInit=0  CountStep=1  CountMax=15  CountFromType=Initial value  CountFrom=0  CountResetPort=off  CountLoadPort=off  CountEnbPort=off  CountDirPort=off  CountHitOutputPort=off  CountDataType=Unsigned  CountWordLen=4  CountFracLen=0  CountSampTime=1.953125e-06
  out0 : Outport  OutDataTypeStr=fixdt(0,4,0,'DataTypeOverride', 'Off')  PortDimensions=1  SampleTime=1.953125e-06  InitialOutput=0
  wires:
  ctr_0_15/1 -> out0/1

== system gm_HFMA_4B_1_5_9_13/Subsystem/HFMA13/crp_temp_shared6/Serializer_Subnetwork ==
  in0 : Inport  OutDataTypeStr=fixdt(1,18,0,'DataTypeOverride', 'Off')  PortDimensions=[16]  SampleTime=1.953125e-06
  in1 : Inport  Port=2  OutDataTypeStr=fixdt(0,4,0,'DataTypeOverride', 'Off')  PortDimensions=1  SampleTime=1.953125e-06
  ratechange_splitcomp : Demux  Outputs=16
  splitcomp_multiport : MultiPortSwitch  DataPortOrder=Zero-based contiguous  Inputs=16  DiagnosticForDefault=None  zeroidx=on  OutDataTypeStr=fixdt(1, 18, 0)  SampleTime=1.953125e-06  SaturateOnIntegerOverflow=off  InputSameDT=off
  out0 : Outport  OutDataTypeStr=fixdt(1,18,0,'DataTypeOverride', 'Off')  PortDimensions=1  SampleTime=1.953125e-06
  wires:
  in0/1 -> ratechange_splitcomp/1
  in1/1 -> splitcomp_multiport/1
  ratechange_splitcomp/2 -> splitcomp_multiport/3
  ratechange_splitcomp/1 -> splitcomp_multiport/2
  ratechange_splitcomp/10 -> splitcomp_multiport/11
  ratechange_splitcomp/8 -> splitcomp_multiport/9
  ratechange_splitcomp/4 -> splitcomp_multiport/5
  ratechange_splitcomp/6 -> splitcomp_multiport/7
  ratechange_splitcomp/9 -> splitcomp_multiport/10
  ratechange_splitcomp/7 -> splitcomp_multiport/8
  ratechange_splitcomp/3 -> splitcomp_multiport/4
  ratechange_splitcomp/5 -> splitcomp_multiport/6
  ratechange_splitcomp/15 -> splitcomp_multiport/16
  ratechange_splitcomp/13 -> splitcomp_multiport/14
  ratechange_splitcomp/11 -> splitcomp_multiport/12
  ratechange_splitcomp/16 -> splitcomp_multiport/17
  ratechange_splitcomp/14 -> splitcomp_multiport/15
  ratechange_splitcomp/12 -> splitcomp_multiport/13
  splitcomp_multiport/1 -> out0/1

== system gm_HFMA_4B_1_5_9_13/Subsystem/HFMA13/crp_temp_shared6/Serializer_Subnetwork1 ==
  in0 : Inport  OutDataTypeStr=fixdt(1,18,0,'DataTypeOverride', 'Off')  PortDimensions=[16]  SampleTime=1.953125e-06
  in1 : Inport  Port=2  OutDataTypeStr=fixdt(0,4,0,'DataTypeOverride', 'Off')  PortDimensions=1  SampleTime=1.953125e-06
  ratechange_splitcomp : Demux  Outputs=16
  splitcomp_multiport : MultiPortSwitch  DataPortOrder=Zero-based contiguous  Inputs=16  DiagnosticForDefault=None  zeroidx=on  OutDataTypeStr=fixdt(1, 18, 0)  SampleTime=1.953125e-06  SaturateOnIntegerOverflow=off  InputSameDT=off
  out0 : Outport  OutDataTypeStr=fixdt(1,18,0,'DataTypeOverride', 'Off')  PortDimensions=1  SampleTime=1.953125e-06
  wires:
  in1/1 -> splitcomp_multiport/1
  in0/1 -> ratechange_splitcomp/1
  ratechange_splitcomp/1 -> splitcomp_multiport/2
  ratechange_splitcomp/3 -> splitcomp_multiport/4
  ratechange_splitcomp/2 -> splitcomp_multiport/3
  ratechange_splitcomp/4 -> splitcomp_multiport/5
  ratechange_splitcomp/6 -> splitcomp_multiport/7
  ratechange_splitcomp/7 -> splitcomp_multiport/8
  ratechange_splitcomp/5 -> splitcomp_multiport/6
  ratechange_splitcomp/8 -> splitcomp_multiport/9
  ratechange_splitcomp/9 -> splitcomp_multiport/10
  ratechange_splitcomp/16 -> splitcomp_multiport/17
  ratechange_splitcomp/14 -> splitcomp_multiport/15
  ratechange_splitcomp/12 -> splitcomp_multiport/13
  ratechange_splitcomp/10 -> splitcomp_multiport/11
  ratechange_splitcomp/15 -> splitcomp_multiport/16
  ratechange_splitcomp/13 -> splitcomp_multiport/14
  ratechange_splitcomp/11 -> splitcomp_multiport/12
  splitcomp_multiport/1 -> out0/1

== system gm_HFMA_4B_1_5_9_13/Subsystem/HFMA13/crp_temp_shared6/counter ==
  globalSchedule : EnablePort  OutDataTypeStr=boolean
  ctr_0_15 : hdlsllib/Sources/HDL Counter  CountType=Count limited  CountInit=0  CountStep=1  CountMax=15  CountFromType=Initial value  CountFrom=0  CountResetPort=off  CountLoadPort=off  CountEnbPort=off  CountDirPort=off  CountHitOutputPort=off  CountDataType=Unsigned  CountWordLen=4  CountFracLen=0  CountSampTime=1.953125e-06
  out0 : Outport  OutDataTypeStr=fixdt(0,4,0,'DataTypeOverride', 'Off')  PortDimensions=1  SampleTime=1.953125e-06  InitialOutput=0
  wires:
  ctr_0_15/1 -> out0/1

== system gm_HFMA_4B_1_5_9_13/Subsystem/HFMA13/crp_temp_shared7/Serializer_Subnetwork ==
  in0 : Inport  OutDataTypeStr=fixdt(1,32,28,'DataTypeOverride', 'Off')  PortDimensions=[2]  SampleTime=1.953125e-06
  in1 : Inport  Port=2  OutDataTypeStr=fixdt(0,1,0,'DataTypeOverride', 'Off')  PortDimensions=1  SampleTime=1.953125e-06
  ratechange_splitcomp : Demux  Outputs=2
  splitcomp_multiport : MultiPortSwitch  DataPortOrder=Zero-based contiguous  Inputs=2  DiagnosticForDefault=None  zeroidx=on  OutDataTypeStr=fixdt(1, 32, 28)  SampleTime=1.953125e-06  SaturateOnIntegerOverflow=off  InputSameDT=off
  out0 : Outport  OutDataTypeStr=fixdt(1,32,28,'DataTypeOverride', 'Off')  PortDimensions=1  SampleTime=1.953125e-06
  wires:
  in0/1 -> ratechange_splitcomp/1
  in1/1 -> splitcomp_multiport/1
  ratechange_splitcomp/2 -> splitcomp_multiport/3
  ratechange_splitcomp/1 -> splitcomp_multiport/2
  splitcomp_multiport/1 -> out0/1

== system gm_HFMA_4B_1_5_9_13/Subsystem/HFMA13/crp_temp_shared7/Serializer_Subnetwork1 ==
  in0 : Inport  OutDataTypeStr=fixdt(1,32,28,'DataTypeOverride', 'Off')  PortDimensions=[2]  SampleTime=1.953125e-06
  in1 : Inport  Port=2  OutDataTypeStr=fixdt(0,1,0,'DataTypeOverride', 'Off')  PortDimensions=1  SampleTime=1.953125e-06
  ratechange_splitcomp : Demux  Outputs=2
  splitcomp_multiport : MultiPortSwitch  DataPortOrder=Zero-based contiguous  Inputs=2  DiagnosticForDefault=None  zeroidx=on  OutDataTypeStr=fixdt(1, 32, 28)  SampleTime=1.953125e-06  SaturateOnIntegerOverflow=off  InputSameDT=off
  out0 : Outport  OutDataTypeStr=fixdt(1,32,28,'DataTypeOverride', 'Off')  PortDimensions=1  SampleTime=1.953125e-06
  wires:
  splitcomp_multiport/1 -> out0/1
  in0/1 -> ratechange_splitcomp/1
  in1/1 -> splitcomp_multiport/1
  ratechange_splitcomp/2 -> splitcomp_multiport/3
  ratechange_splitcomp/1 -> splitcomp_multiport/2

== system gm_HFMA_4B_1_5_9_13/Subsystem/HFMA13/crp_temp_shared7/counter ==
  globalSchedule : EnablePort  OutDataTypeStr=boolean
  ctr_0_1 : hdlsllib/Sources/HDL Counter  CountType=Count limited  CountInit=0  CountStep=1  CountMax=1  CountFromType=Initial value  CountFrom=0  CountResetPort=off  CountLoadPort=off  CountEnbPort=off  CountDirPort=off  CountHitOutputPort=off  CountDataType=Unsigned  CountWordLen=1  CountFracLen=0  CountSampTime=1.953125e-06
  out0 : Outport  OutDataTypeStr=fixdt(0,1,0,'DataTypeOverride', 'Off')  PortDimensions=1  SampleTime=1.953125e-06  InitialOutput=0
  wires:
  ctr_0_1/1 -> out0/1

== system gm_HFMA_4B_1_5_9_13/Subsystem/HFMA13/crp_temp_shared8/Serializer_Subnetwork ==
  in0 : Inport  OutDataTypeStr=fixdt(1,18,0,'DataTypeOverride', 'Off')  PortDimensions=[16]  SampleTime=1.953125e-06
  in1 : Inport  Port=2  OutDataTypeStr=fixdt(0,4,0,'DataTypeOverride', 'Off')  PortDimensions=1  SampleTime=1.953125e-06
  ratechange_splitcomp : Demux  Outputs=16
  splitcomp_multiport : MultiPortSwitch  DataPortOrder=Zero-based contiguous  Inputs=16  DiagnosticForDefault=None  zeroidx=on  OutDataTypeStr=fixdt(1, 18, 0)  SampleTime=1.953125e-06  SaturateOnIntegerOverflow=off  InputSameDT=off
  out0 : Outport  OutDataTypeStr=fixdt(1,18,0,'DataTypeOverride', 'Off')  PortDimensions=1  SampleTime=1.953125e-06
  wires:
  in0/1 -> ratechange_splitcomp/1
  in1/1 -> splitcomp_multiport/1
  ratechange_splitcomp/2 -> splitcomp_multiport/3
  ratechange_splitcomp/4 -> splitcomp_multiport/5
  ratechange_splitcomp/6 -> splitcomp_multiport/7
  ratechange_splitcomp/7 -> splitcomp_multiport/8
  ratechange_splitcomp/1 -> splitcomp_multiport/2
  ratechange_splitcomp/3 -> splitcomp_multiport/4
  ratechange_splitcomp/5 -> splitcomp_multiport/6
  ratechange_splitcomp/14 -> splitcomp_multiport/15
  ratechange_splitcomp/12 -> splitcomp_multiport/13
  ratechange_splitcomp/10 -> splitcomp_multiport/11
  ratechange_splitcomp/8 -> splitcomp_multiport/9
  ratechange_splitcomp/15 -> splitcomp_multiport/16
  ratechange_splitcomp/13 -> splitcomp_multiport/14
  ratechange_splitcomp/11 -> splitcomp_multiport/12
  ratechange_splitcomp/9 -> splitcomp_multiport/10
  splitcomp_multiport/1 -> out0/1
  ratechange_splitcomp/16 -> splitcomp_multiport/17

== system gm_HFMA_4B_1_5_9_13/Subsystem/HFMA13/crp_temp_shared8/Serializer_Subnetwork1 ==
  in0 : Inport  OutDataTypeStr=fixdt(1,18,0,'DataTypeOverride', 'Off')  PortDimensions=[16]  SampleTime=1.953125e-06
  in1 : Inport  Port=2  OutDataTypeStr=fixdt(0,4,0,'DataTypeOverride', 'Off')  PortDimensions=1  SampleTime=1.953125e-06
  ratechange_splitcomp : Demux  Outputs=16
  splitcomp_multiport : MultiPortSwitch  DataPortOrder=Zero-based contiguous  Inputs=16  DiagnosticForDefault=None  zeroidx=on  OutDataTypeStr=fixdt(1, 18, 0)  SampleTime=1.953125e-06  SaturateOnIntegerOverflow=off  InputSameDT=off
  out0 : Outport  OutDataTypeStr=fixdt(1,18,0,'DataTypeOverride', 'Off')  PortDimensions=1  SampleTime=1.953125e-06
  wires:
  in0/1 -> ratechange_splitcomp/1
  in1/1 -> splitcomp_multiport/1
  ratechange_splitcomp/2 -> splitcomp_multiport/3
  ratechange_splitcomp/4 -> splitcomp_multiport/5
  ratechange_splitcomp/6 -> splitcomp_multiport/7
  ratechange_splitcomp/7 -> splitcomp_multiport/8
  ratechange_splitcomp/1 -> splitcomp_multiport/2
  ratechange_splitcomp/3 -> splitcomp_multiport/4
  ratechange_splitcomp/5 -> splitcomp_multiport/6
  ratechange_splitcomp/8 -> splitcomp_multiport/9
  ratechange_splitcomp/9 -> splitcomp_multiport/10
  ratechange_splitcomp/12 -> splitcomp_multiport/13
  ratechange_splitcomp/10 -> splitcomp_multiport/11
  ratechange_splitcomp/13 -> splitcomp_multiport/14
  ratechange_splitcomp/11 -> splitcomp_multiport/12
  ratechange_splitcomp/16 -> splitcomp_multiport/17
  ratechange_splitcomp/14 -> splitcomp_multiport/15
  ratechange_splitcomp/15 -> splitcomp_multiport/16
  splitcomp_multiport/1 -> out0/1

== system gm_HFMA_4B_1_5_9_13/Subsystem/HFMA13/crp_temp_shared8/counter ==
  globalSchedule : EnablePort  OutDataTypeStr=boolean
  ctr_0_15 : hdlsllib/Sources/HDL Counter  CountType=Count limited  CountInit=0  CountStep=1  CountMax=15  CountFromType=Initial value  CountFrom=0  CountResetPort=off  CountLoadPort=off  CountEnbPort=off  CountDirPort=off  CountHitOutputPort=off  CountDataType=Unsigned  CountWordLen=4  CountFracLen=0  CountSampTime=1.953125e-06
  out0 : Outport  OutDataTypeStr=fixdt(0,4,0,'DataTypeOverride', 'Off')  PortDimensions=1  SampleTime=1.953125e-06  InitialOutput=0
  wires:
  ctr_0_15/1 -> out0/1

== system gm_HFMA_4B_1_5_9_13/Subsystem/HFMA13/crp_temp_shared9/Serializer_Subnetwork ==
  in0 : Inport  OutDataTypeStr=fixdt(1,18,16,'DataTypeOverride', 'Off')  PortDimensions=[2]  SampleTime=1.953125e-06
  in1 : Inport  Port=2  OutDataTypeStr=fixdt(0,1,0,'DataTypeOverride', 'Off')  PortDimensions=1  SampleTime=1.953125e-06
  ratechange_splitcomp : Demux  Outputs=2
  splitcomp_multiport : MultiPortSwitch  DataPortOrder=Zero-based contiguous  Inputs=2  DiagnosticForDefault=None  zeroidx=on  OutDataTypeStr=fixdt(1, 18, 16)  SampleTime=1.953125e-06  SaturateOnIntegerOverflow=off  InputSameDT=off
  out0 : Outport  OutDataTypeStr=fixdt(1,18,16,'DataTypeOverride', 'Off')  PortDimensions=1  SampleTime=1.953125e-06
  wires:
  in0/1 -> ratechange_splitcomp/1
  in1/1 -> splitcomp_multiport/1
  ratechange_splitcomp/2 -> splitcomp_multiport/3
  ratechange_splitcomp/1 -> splitcomp_multiport/2
  splitcomp_multiport/1 -> out0/1

== system gm_HFMA_4B_1_5_9_13/Subsystem/HFMA13/crp_temp_shared9/Serializer_Subnetwork1 ==
  in0 : Inport  OutDataTypeStr=fixdt(1,18,16,'DataTypeOverride', 'Off')  PortDimensions=[2]  SampleTime=1.953125e-06
  in1 : Inport  Port=2  OutDataTypeStr=fixdt(0,1,0,'DataTypeOverride', 'Off')  PortDimensions=1  SampleTime=1.953125e-06
  ratechange_splitcomp : Demux  Outputs=2
  splitcomp_multiport : MultiPortSwitch  DataPortOrder=Zero-based contiguous  Inputs=2  DiagnosticForDefault=None  zeroidx=on  OutDataTypeStr=fixdt(1, 18, 16)  SampleTime=1.953125e-06  SaturateOnIntegerOverflow=off  InputSameDT=off
  out0 : Outport  OutDataTypeStr=fixdt(1,18,16,'DataTypeOverride', 'Off')  PortDimensions=1  SampleTime=1.953125e-06
  wires:
  in0/1 -> ratechange_splitcomp/1
  in1/1 -> splitcomp_multiport/1
  ratechange_splitcomp/2 -> splitcomp_multiport/3
  ratechange_splitcomp/1 -> splitcomp_multiport/2
  splitcomp_multiport/1 -> out0/1

== system gm_HFMA_4B_1_5_9_13/Subsystem/HFMA13/crp_temp_shared9/counter ==
  globalSchedule : EnablePort  OutDataTypeStr=boolean
  ctr_0_1 : hdlsllib/Sources/HDL Counter  CountType=Count limited  CountInit=0  CountStep=1  CountMax=1  CountFromType=Initial value  CountFrom=0  CountResetPort=off  CountLoadPort=off  CountEnbPort=off  CountDirPort=off  CountHitOutputPort=off  CountDataType=Unsigned  CountWordLen=1  CountFracLen=0  CountSampTime=1.953125e-06
  out0 : Outport  OutDataTypeStr=fixdt(0,1,0,'DataTypeOverride', 'Off')  PortDimensions=1  SampleTime=1.953125e-06  InitialOutput=0
  wires:
  ctr_0_1/1 -> out0/1

== system gm_HFMA_4B_1_5_9_13/Subsystem/HFMA5/crp_temp_shared/Product3_out1_bypass ==
  in0 : Inport  OutDataTypeStr=fixdt(1,51,0,'DataTypeOverride', 'Off')  PortDimensions=1  SampleTime=1.953125e-06
  in1 : Inport  Port=2  OutDataTypeStr=boolean  PortDimensions=1  SampleTime=1.953125e-06
  Product3_out1_enb : Switch  Criteria=u2 ~= 0  OutDataTypeStr=fixdt(1, 51, 0)  SampleTime=1.953125e-06  SaturateOnIntegerOverflow=off  InputSameDT=off
  Product3_out1_state : Delay  DelayLength=1  InitialCondition=0  SampleTime=1.953125e-06
  out0 : Outport  OutDataTypeStr=fixdt(1,51,0,'DataTypeOverride', 'Off')  PortDimensions=1  SampleTime=1.953125e-06
  wires:
  in1/1 -> Product3_out1_enb/2
  in0/1 -> Product3_out1_enb/1
  Product3_out1_state/1 -> Product3_out1_enb/3
  Product3_out1_enb/1 -> Product3_out1_state/1, out0/1
